simulink model "FBR25_model_4_rotating_tyres_with_ground_no_contact"  (R2026a)
settings: Solver=VariableStepAuto  StopTime=5
model workspace: external: MATLAB File /Users/janabauer/Desktop/LTS-test/models/FBR25forVD_DataFile1.m (data not in the file)
undefined symbols (not defined in the file or in its folder): smiData, X, Y, Z
libraries: sm_lib x832, nesl_utility x5, simulink x1
(part 13 of 13)

== system FBR25_model_4_rotating_tyres_with_ground_no_contact/FBR25_VD_1_RIGID/FBR25_VD_0300_STEERING_Computurtle_3_1_RIGID/FBR25_VD_33_00_1_RIGID/FBR25_VD_33_06_1_RIGID ==
  ReferenceFrame : sm_lib/Frames and Transforms/Reference Frame
  Solid : sm_lib/Body Elements/File Solid  ExtGeomFileName=FBR25-VD-33-06_Default_sldprt.STEP  UnitType=FromFile  ExtGeomFileUnits=m  StepReaderType=HEX  ExportConvexHullGeometry=off  InertiaType=Custom  BasedOnType=DensityFromFile  Density=1000  DensityUnits=kg/m^3  Mass=smiData.Solid(89).mass  MassUnits=kg  CenterOfMass=smiData.Solid(89).CoM  CenterOfMassUnits=mm  MomentsOfInertia=smiData.Solid(89).MoI  MomentsOfInertiaUnits=kg*mm^2  ProductsOfInertia=smiData.Solid(89).PoI  ProductsOfInertiaUnits=kg*mm^2  GraphicType=FromGeometry  MarkerShape=Sphere  MarkerSize=10  GraphicVisPropType=SimpleVisualProperties  GraphicDiffuseColor=smiData.Solid(89).color  GraphicOpacity=smiData.Solid(89).opacity  GraphicSpecularColor=[0.5 0.5 0.5 1.0]  GraphicAmbientColor=[0.15 0.15 0.15 1.0]  GraphicEmissiveColor=[0.0 0.0 0.0 1.0]  GraphicShininess=75  DoExposeReferenceFrame=on  SerializedFrames=<Frames/>
  F : PMIOPort  Side=Left
  connections:
  Solid/RConn1 -- ReferenceFrame/RConn1 -- F/RConn1

== system FBR25_model_4_rotating_tyres_with_ground_no_contact/FBR25_VD_1_RIGID/FBR25_VD_0300_STEERING_Computurtle_3_1_RIGID/FBR25_VD_33_00_1_RIGID/FBR25_VD_33_06_2_RIGID ==
  ReferenceFrame : sm_lib/Frames and Transforms/Reference Frame
  Solid : sm_lib/Body Elements/File Solid  ExtGeomFileName=FBR25-VD-33-06_Default_sldprt.STEP  UnitType=FromFile  ExtGeomFileUnits=m  StepReaderType=HEX  ExportConvexHullGeometry=off  InertiaType=Custom  BasedOnType=DensityFromFile  Density=1000  DensityUnits=kg/m^3  Mass=smiData.Solid(89).mass  MassUnits=kg  CenterOfMass=smiData.Solid(89).CoM  CenterOfMassUnits=mm  MomentsOfInertia=smiData.Solid(89).MoI  MomentsOfInertiaUnits=kg*mm^2  ProductsOfInertia=smiData.Solid(89).PoI  ProductsOfInertiaUnits=kg*mm^2  GraphicType=FromGeometry  MarkerShape=Sphere  MarkerSize=10  GraphicVisPropType=SimpleVisualProperties  GraphicDiffuseColor=smiData.Solid(89).color  GraphicOpacity=smiData.Solid(89).opacity  GraphicSpecularColor=[0.5 0.5 0.5 1.0]  GraphicAmbientColor=[0.15 0.15 0.15 1.0]  GraphicEmissiveColor=[0.0 0.0 0.0 1.0]  GraphicShininess=75  DoExposeReferenceFrame=on  SerializedFrames=<Frames/>
  F : PMIOPort  Side=Left
  connections:
  Solid/RConn1 -- ReferenceFrame/RConn1 -- F/RConn1

== system FBR25_model_4_rotating_tyres_with_ground_no_contact/FBR25_VD_1_RIGID/FBR25_VD_0300_STEERING_Computurtle_3_1_RIGID/FBR25_VD_33_00_1_RIGID/Part3_1_RIGID ==
  ReferenceFrame : sm_lib/Frames and Transforms/Reference Frame
  Solid : sm_lib/Body Elements/File Solid  ExtGeomFileName=Part3_Default_sldprt.STEP  UnitType=FromFile  ExtGeomFileUnits=m  StepReaderType=HEX  ExportConvexHullGeometry=off  InertiaType=Custom  BasedOnType=DensityFromFile  Density=1000  DensityUnits=kg/m^3  Mass=smiData.Solid(90).mass  MassUnits=kg  CenterOfMass=smiData.Solid(90).CoM  CenterOfMassUnits=mm  MomentsOfInertia=smiData.Solid(90).MoI  MomentsOfInertiaUnits=kg*mm^2  ProductsOfInertia=smiData.Solid(90).PoI  ProductsOfInertiaUnits=kg*mm^2  GraphicType=FromGeometry  MarkerShape=Sphere  MarkerSize=10  GraphicVisPropType=SimpleVisualProperties  GraphicDiffuseColor=smiData.Solid(90).color  GraphicOpacity=smiData.Solid(90).opacity  GraphicSpecularColor=[0.5 0.5 0.5 1.0]  GraphicAmbientColor=[0.15 0.15 0.15 1.0]  GraphicEmissiveColor=[0.0 0.0 0.0 1.0]  GraphicShininess=75  DoExposeReferenceFrame=on  SerializedFrames=<Frames/>
  F : PMIOPort  Side=Left
  connections:
  Solid/RConn1 -- ReferenceFrame/RConn1 -- F/RConn1

== system FBR25_model_4_rotating_tyres_with_ground_no_contact/FBR25_VD_1_RIGID/FBR25_VD_0300_STEERING_Computurtle_3_1_RIGID/FBR25_VD_33_00_1_RIGID/Part3_2_RIGID ==
  ReferenceFrame : sm_lib/Frames and Transforms/Reference Frame
  Solid : sm_lib/Body Elements/File Solid  ExtGeomFileName=Part3_Default_sldprt.STEP  UnitType=FromFile  ExtGeomFileUnits=m  StepReaderType=HEX  ExportConvexHullGeometry=off  InertiaType=Custom  BasedOnType=DensityFromFile  Density=1000  DensityUnits=kg/m^3  Mass=smiData.Solid(90).mass  MassUnits=kg  CenterOfMass=smiData.Solid(90).CoM  CenterOfMassUnits=mm  MomentsOfInertia=smiData.Solid(90).MoI  MomentsOfInertiaUnits=kg*mm^2  ProductsOfInertia=smiData.Solid(90).PoI  ProductsOfInertiaUnits=kg*mm^2  GraphicType=FromGeometry  MarkerShape=Sphere  MarkerSize=10  GraphicVisPropType=SimpleVisualProperties  GraphicDiffuseColor=smiData.Solid(90).color  GraphicOpacity=smiData.Solid(90).opacity  GraphicSpecularColor=[0.5 0.5 0.5 1.0]  GraphicAmbientColor=[0.15 0.15 0.15 1.0]  GraphicEmissiveColor=[0.0 0.0 0.0 1.0]  GraphicShininess=75  DoExposeReferenceFrame=on  SerializedFrames=<Frames/>
  F : PMIOPort  Side=Left
  connections:
  Solid/RConn1 -- ReferenceFrame/RConn1 -- F/RConn1

== system FBR25_model_4_rotating_tyres_with_ground_no_contact/FBR25_VD_1_RIGID/FBR25_VD_0300_STEERING_Computurtle_3_1_RIGID/FBR25_VD_33_00_1_RIGID/SPACER_M8_MISALIGNMENT_1_RIGID ==
  ReferenceFrame : sm_lib/Frames and Transforms/Reference Frame
  Solid : sm_lib/Body Elements/File Solid  ExtGeomFileName=SPACER - M8 MISALIGNMENT_Default_sldprt.STEP  UnitType=FromFile  ExtGeomFileUnits=m  StepReaderType=HEX  ExportConvexHullGeometry=off  InertiaType=Custom  BasedOnType=DensityFromFile  Density=1000  DensityUnits=kg/m^3  Mass=smiData.Solid(23).mass  MassUnits=kg  CenterOfMass=smiData.Solid(23).CoM  CenterOfMassUnits=mm  MomentsOfInertia=smiData.Solid(23).MoI  MomentsOfInertiaUnits=kg*mm^2  ProductsOfInertia=smiData.Solid(23).PoI  ProductsOfInertiaUnits=kg*mm^2  GraphicType=FromGeometry  MarkerShape=Sphere  MarkerSize=10  GraphicVisPropType=SimpleVisualProperties  GraphicDiffuseColor=smiData.Solid(23).color  GraphicOpacity=smiData.Solid(23).opacity  GraphicSpecularColor=[0.5 0.5 0.5 1.0]  GraphicAmbientColor=[0.15 0.15 0.15 1.0]  GraphicEmissiveColor=[0.0 0.0 0.0 1.0]  GraphicShininess=75  DoExposeReferenceFrame=on  SerializedFrames=<Frames/>
  F : PMIOPort  Side=Left
  connections:
  Solid/RConn1 -- ReferenceFrame/RConn1 -- F/RConn1

== system FBR25_model_4_rotating_tyres_with_ground_no_contact/FBR25_VD_1_RIGID/FBR25_VD_0300_STEERING_Computurtle_3_1_RIGID/FBR25_VD_33_00_1_RIGID/SPACER_M8_MISALIGNMENT_2_RIGID ==
  ReferenceFrame : sm_lib/Frames and Transforms/Reference Frame
  Solid : sm_lib/Body Elements/File Solid  ExtGeomFileName=SPACER - M8 MISALIGNMENT_Default_sldprt.STEP  UnitType=FromFile  ExtGeomFileUnits=m  StepReaderType=HEX  ExportConvexHullGeometry=off  InertiaType=Custom  BasedOnType=DensityFromFile  Density=1000  DensityUnits=kg/m^3  Mass=smiData.Solid(23).mass  MassUnits=kg  CenterOfMass=smiData.Solid(23).CoM  CenterOfMassUnits=mm  MomentsOfInertia=smiData.Solid(23).MoI  MomentsOfInertiaUnits=kg*mm^2  ProductsOfInertia=smiData.Solid(23).PoI  ProductsOfInertiaUnits=kg*mm^2  GraphicType=FromGeometry  MarkerShape=Sphere  MarkerSize=10  GraphicVisPropType=SimpleVisualProperties  GraphicDiffuseColor=smiData.Solid(23).color  GraphicOpacity=smiData.Solid(23).opacity  GraphicSpecularColor=[0.5 0.5 0.5 1.0]  GraphicAmbientColor=[0.15 0.15 0.15 1.0]  GraphicEmissiveColor=[0.0 0.0 0.0 1.0]  GraphicShininess=75  DoExposeReferenceFrame=on  SerializedFrames=<Frames/>
  F : PMIOPort  Side=Left
  connections:
  Solid/RConn1 -- ReferenceFrame/RConn1 -- F/RConn1

== system FBR25_model_4_rotating_tyres_with_ground_no_contact/FBR25_VD_1_RIGID/FBR25_VD_0300_STEERING_Computurtle_3_1_RIGID/FBR25_VD_33_00_1_RIGID/SPACER_M8_MISALIGNMENT_3_RIGID ==
  ReferenceFrame : sm_lib/Frames and Transforms/Reference Frame
  Solid : sm_lib/Body Elements/File Solid  ExtGeomFileName=SPACER - M8 MISALIGNMENT_Default_sldprt.STEP  UnitType=FromFile  ExtGeomFileUnits=m  StepReaderType=HEX  ExportConvexHullGeometry=off  InertiaType=Custom  BasedOnType=DensityFromFile  Density=1000  DensityUnits=kg/m^3  Mass=smiData.Solid(23).mass  MassUnits=kg  CenterOfMass=smiData.Solid(23).CoM  CenterOfMassUnits=mm  MomentsOfInertia=smiData.Solid(23).MoI  MomentsOfInertiaUnits=kg*mm^2  ProductsOfInertia=smiData.Solid(23).PoI  ProductsOfInertiaUnits=kg*mm^2  GraphicType=FromGeometry  MarkerShape=Sphere  MarkerSize=10  GraphicVisPropType=SimpleVisualProperties  GraphicDiffuseColor=smiData.Solid(23).color  GraphicOpacity=smiData.Solid(23).opacity  GraphicSpecularColor=[0.5 0.5 0.5 1.0]  GraphicAmbientColor=[0.15 0.15 0.15 1.0]  GraphicEmissiveColor=[0.0 0.0 0.0 1.0]  GraphicShininess=75  DoExposeReferenceFrame=on  SerializedFrames=<Frames/>
  F : PMIOPort  Side=Left
  connections:
  Solid/RConn1 -- ReferenceFrame/RConn1 -- F/RConn1

== system FBR25_model_4_rotating_tyres_with_ground_no_contact/FBR25_VD_1_RIGID/FBR25_VD_0300_STEERING_Computurtle_3_1_RIGID/FBR25_VD_33_00_1_RIGID/SPACER_M8_MISALIGNMENT_4_RIGID ==
  ReferenceFrame : sm_lib/Frames and Transforms/Reference Frame
  Solid : sm_lib/Body Elements/File Solid  ExtGeomFileName=SPACER - M8 MISALIGNMENT_Default_sldprt.STEP  UnitType=FromFile  ExtGeomFileUnits=m  StepReaderType=HEX  ExportConvexHullGeometry=off  InertiaType=Custom  BasedOnType=DensityFromFile  Density=1000  DensityUnits=kg/m^3  Mass=smiData.Solid(23).mass  MassUnits=kg  CenterOfMass=smiData.Solid(23).CoM  CenterOfMassUnits=mm  MomentsOfInertia=smiData.Solid(23).MoI  MomentsOfInertiaUnits=kg*mm^2  ProductsOfInertia=smiData.Solid(23).PoI  ProductsOfInertiaUnits=kg*mm^2  GraphicType=FromGeometry  MarkerShape=Sphere  MarkerSize=10  GraphicVisPropType=SimpleVisualProperties  GraphicDiffuseColor=smiData.Solid(23).color  GraphicOpacity=smiData.Solid(23).opacity  GraphicSpecularColor=[0.5 0.5 0.5 1.0]  GraphicAmbientColor=[0.15 0.15 0.15 1.0]  GraphicEmissiveColor=[0.0 0.0 0.0 1.0]  GraphicShininess=75  DoExposeReferenceFrame=on  SerializedFrames=<Frames/>
  F : PMIOPort  Side=Left
  connections:
  Solid/RConn1 -- ReferenceFrame/RConn1 -- F/RConn1

== system FBR25_model_4_rotating_tyres_with_ground_no_contact/FBR25_VD_1_RIGID/FBR25_VD_0000_WISHBONES_1_RIGID/FBR25_VD_0010_WB_F_U_1_RIGID/FBR25_VD_00_14_NH_01_1_RIGID/FBR25_VD_00_14_NH_01_ball_1_RIGID ==
  ReferenceFrame : sm_lib/Frames and Transforms/Reference Frame
  Solid : sm_lib/Body Elements/File Solid  ExtGeomFileName=FBR25-VD-00-14-NH-01 ball_Default_sldprt.STEP  UnitType=FromFile  ExtGeomFileUnits=m  StepReaderType=HEX  ExportConvexHullGeometry=off  InertiaType=Custom  BasedOnType=DensityFromFile  Density=1000  DensityUnits=kg/m^3  Mass=smiData.Solid(30).mass  MassUnits=kg  CenterOfMass=smiData.Solid(30).CoM  CenterOfMassUnits=mm  MomentsOfInertia=smiData.Solid(30).MoI  MomentsOfInertiaUnits=kg*mm^2  ProductsOfInertia=smiData.Solid(30).PoI  ProductsOfInertiaUnits=kg*mm^2  GraphicType=FromGeometry  MarkerShape=Sphere  MarkerSize=10  GraphicVisPropType=SimpleVisualProperties  GraphicDiffuseColor=smiData.Solid(30).color  GraphicOpacity=smiData.Solid(30).opacity  GraphicSpecularColor=[0.5 0.5 0.5 1.0]  GraphicAmbientColor=[0.15 0.15 0.15 1.0]  GraphicEmissiveColor=[0.0 0.0 0.0 1.0]  GraphicShininess=75  DoExposeReferenceFrame=on  SerializedFrames=<Frames/>
  F : PMIOPort  Side=Left
  connections:
  Solid/RConn1 -- ReferenceFrame/RConn1 -- F/RConn1

== system FBR25_model_4_rotating_tyres_with_ground_no_contact/FBR25_VD_1_RIGID/FBR25_VD_0000_WISHBONES_1_RIGID/FBR25_VD_0010_WB_F_U_1_RIGID/FBR25_VD_00_14_NH_01_1_RIGID/FBR25_VD_00_14_NH_01_casing_1_RIGID ==
  ReferenceFrame : sm_lib/Frames and Transforms/Reference Frame
  Solid : sm_lib/Body Elements/File Solid  ExtGeomFileName=FBR25-VD-00-14-NH-01 casing_Default_sldprt.STEP  UnitType=FromFile  ExtGeomFileUnits=m  StepReaderType=HEX  ExportConvexHullGeometry=off  InertiaType=Custom  BasedOnType=DensityFromFile  Density=1000  DensityUnits=kg/m^3  Mass=smiData.Solid(31).mass  MassUnits=kg  CenterOfMass=smiData.Solid(31).CoM  CenterOfMassUnits=mm  MomentsOfInertia=smiData.Solid(31).MoI  MomentsOfInertiaUnits=kg*mm^2  ProductsOfInertia=smiData.Solid(31).PoI  ProductsOfInertiaUnits=kg*mm^2  GraphicType=FromGeometry  MarkerShape=Sphere  MarkerSize=10  GraphicVisPropType=SimpleVisualProperties  GraphicDiffuseColor=smiData.Solid(31).color  GraphicOpacity=smiData.Solid(31).opacity  GraphicSpecularColor=[0.5 0.5 0.5 1.0]  GraphicAmbientColor=[0.15 0.15 0.15 1.0]  GraphicEmissiveColor=[0.0 0.0 0.0 1.0]  GraphicShininess=75  DoExposeReferenceFrame=on  SerializedFrames=<Frames/>
  F : PMIOPort  Side=Left
  connections:
  Solid/RConn1 -- ReferenceFrame/RConn1 -- F/RConn1

== system FBR25_model_4_rotating_tyres_with_ground_no_contact/FBR25_VD_1_RIGID/FBR25_VD_0000_WISHBONES_1_RIGID/FBR25_VD_0020_1_RIGID/FBR25_VD_00_24_NH_01_1_RIGID/FBR25_VD_00_24_NH_01_ball_1_RIGID ==
  ReferenceFrame : sm_lib/Frames and Transforms/Reference Frame
  Solid : sm_lib/Body Elements/File Solid  ExtGeomFileName=FBR25-VD-00-24-NH-01 - ball_Default_sldprt.STEP  UnitType=FromFile  ExtGeomFileUnits=m  StepReaderType=HEX  ExportConvexHullGeometry=off  InertiaType=Custom  BasedOnType=DensityFromFile  Density=1000  DensityUnits=kg/m^3  Mass=smiData.Solid(49).mass  MassUnits=kg  CenterOfMass=smiData.Solid(49).CoM  CenterOfMassUnits=mm  MomentsOfInertia=smiData.Solid(49).MoI  MomentsOfInertiaUnits=kg*mm^2  ProductsOfInertia=smiData.Solid(49).PoI  ProductsOfInertiaUnits=kg*mm^2  GraphicType=FromGeometry  MarkerShape=Sphere  MarkerSize=10  GraphicVisPropType=SimpleVisualProperties  GraphicDiffuseColor=smiData.Solid(49).color  GraphicOpacity=smiData.Solid(49).opacity  GraphicSpecularColor=[0.5 0.5 0.5 1.0]  GraphicAmbientColor=[0.15 0.15 0.15 1.0]  GraphicEmissiveColor=[0.0 0.0 0.0 1.0]  GraphicShininess=75  DoExposeReferenceFrame=on  SerializedFrames=<Frames/>
  F : PMIOPort  Side=Left
  connections:
  Solid/RConn1 -- ReferenceFrame/RConn1 -- F/RConn1

== system FBR25_model_4_rotating_tyres_with_ground_no_contact/FBR25_VD_1_RIGID/FBR25_VD_0000_WISHBONES_1_RIGID/FBR25_VD_0020_1_RIGID/FBR25_VD_00_24_NH_01_1_RIGID/FBR25_VD_00_24_NH_01_casing_1_RIGID ==
  ReferenceFrame : sm_lib/Frames and Transforms/Reference Frame
  Solid : sm_lib/Body Elements/File Solid  ExtGeomFileName=FBR25-VD-00-24-NH-01 - casing_Default_sldprt.STEP  UnitType=FromFile  ExtGeomFileUnits=m  StepReaderType=HEX  ExportConvexHullGeometry=off  InertiaType=Custom  BasedOnType=DensityFromFile  Density=1000  DensityUnits=kg/m^3  Mass=smiData.Solid(48).mass  MassUnits=kg  CenterOfMass=smiData.Solid(48).CoM  CenterOfMassUnits=mm  MomentsOfInertia=smiData.Solid(48).MoI  MomentsOfInertiaUnits=kg*mm^2  ProductsOfInertia=smiData.Solid(48).PoI  ProductsOfInertiaUnits=kg*mm^2  GraphicType=FromGeometry  MarkerShape=Sphere  MarkerSize=10  GraphicVisPropType=SimpleVisualProperties  GraphicDiffuseColor=smiData.Solid(48).color  GraphicOpacity=smiData.Solid(48).opacity  GraphicSpecularColor=[0.5 0.5 0.5 1.0]  GraphicAmbientColor=[0.15 0.15 0.15 1.0]  GraphicEmissiveColor=[0.0 0.0 0.0 1.0]  GraphicShininess=75  DoExposeReferenceFrame=on  SerializedFrames=<Frames/>
  F : PMIOPort  Side=Left
  connections:
  Solid/RConn1 -- ReferenceFrame/RConn1 -- F/RConn1

== system FBR25_model_4_rotating_tyres_with_ground_no_contact/FBR25_VD_1_RIGID/FBR25_VD_0000_WISHBONES_1_RIGID/FBR25_VD_0020_1_RIGID/MirrorFBR25_VD_00_24_NH_01_2_RIGID/MirrorFBR25_VD_00_24_NH_01_ball_1_RIGID ==
  ReferenceFrame : sm_lib/Frames and Transforms/Reference Frame
  Solid : sm_lib/Body Elements/File Solid  ExtGeomFileName=MirrorFBR25-VD-00-24-NH-01 - ball_Default_sldprt.STEP  UnitType=FromFile  ExtGeomFileUnits=m  StepReaderType=HEX  ExportConvexHullGeometry=off  InertiaType=Custom  BasedOnType=DensityFromFile  Density=1000  DensityUnits=kg/m^3  Mass=smiData.Solid(54).mass  MassUnits=kg  CenterOfMass=smiData.Solid(54).CoM  CenterOfMassUnits=mm  MomentsOfInertia=smiData.Solid(54).MoI  MomentsOfInertiaUnits=kg*mm^2  ProductsOfInertia=smiData.Solid(54).PoI  ProductsOfInertiaUnits=kg*mm^2  GraphicType=FromGeometry  MarkerShape=Sphere  MarkerSize=10  GraphicVisPropType=SimpleVisualProperties  GraphicDiffuseColor=smiData.Solid(54).color  GraphicOpacity=smiData.Solid(54).opacity  GraphicSpecularColor=[0.5 0.5 0.5 1.0]  GraphicAmbientColor=[0.15 0.15 0.15 1.0]  GraphicEmissiveColor=[0.0 0.0 0.0 1.0]  GraphicShininess=75  DoExposeReferenceFrame=on  SerializedFrames=<Frames/>
  F : PMIOPort  Side=Left
  connections:
  Solid/RConn1 -- ReferenceFrame/RConn1 -- F/RConn1

== system FBR25_model_4_rotating_tyres_with_ground_no_contact/FBR25_VD_1_RIGID/FBR25_VD_0000_WISHBONES_1_RIGID/FBR25_VD_0020_1_RIGID/MirrorFBR25_VD_00_24_NH_01_2_RIGID/MirrorFBR25_VD_00_24_NH_01_casing_1_RIGID ==
  ReferenceFrame : sm_lib/Frames and Transforms/Reference Frame
  Solid : sm_lib/Body Elements/File Solid  ExtGeomFileName=MirrorFBR25-VD-00-24-NH-01 - casing_Default_sldprt.STEP  UnitType=FromFile  ExtGeomFileUnits=m  StepReaderType=HEX  ExportConvexHullGeometry=off  InertiaType=Custom  BasedOnType=DensityFromFile  Density=1000  DensityUnits=kg/m^3  Mass=smiData.Solid(53).mass  MassUnits=kg  CenterOfMass=smiData.Solid(53).CoM  CenterOfMassUnits=mm  MomentsOfInertia=smiData.Solid(53).MoI  MomentsOfInertiaUnits=kg*mm^2  ProductsOfInertia=smiData.Solid(53).PoI  ProductsOfInertiaUnits=kg*mm^2  GraphicType=FromGeometry  MarkerShape=Sphere  MarkerSize=10  GraphicVisPropType=SimpleVisualProperties  GraphicDiffuseColor=smiData.Solid(53).color  GraphicOpacity=smiData.Solid(53).opacity  GraphicSpecularColor=[0.5 0.5 0.5 1.0]  GraphicAmbientColor=[0.15 0.15 0.15 1.0]  GraphicEmissiveColor=[0.0 0.0 0.0 1.0]  GraphicShininess=75  DoExposeReferenceFrame=on  SerializedFrames=<Frames/>
  F : PMIOPort  Side=Left
  connections:
  Solid/RConn1 -- ReferenceFrame/RConn1 -- F/RConn1

== system FBR25_model_4_rotating_tyres_with_ground_no_contact/FBR25_VD_1_RIGID/FBR25_VD_0000_WISHBONES_1_RIGID/FBR25_VD_0060_2_RIGID/FBR25_VD_00_64_NH_01_1_RIGID/FBR25_VD_00_64_NH_01_ball_1_RIGID ==
  ReferenceFrame : sm_lib/Frames and Transforms/Reference Frame
  Solid : sm_lib/Body Elements/File Solid  ExtGeomFileName=FBR25-VD-00-64-NH-01 ball_Default_sldprt.STEP  UnitType=FromFile  ExtGeomFileUnits=m  StepReaderType=HEX  ExportConvexHullGeometry=off  InertiaType=Custom  BasedOnType=DensityFromFile  Density=1000  DensityUnits=kg/m^3  Mass=smiData.Solid(41).mass  MassUnits=kg  CenterOfMass=smiData.Solid(41).CoM  CenterOfMassUnits=mm  MomentsOfInertia=smiData.Solid(41).MoI  MomentsOfInertiaUnits=kg*mm^2  ProductsOfInertia=smiData.Solid(41).PoI  ProductsOfInertiaUnits=kg*mm^2  GraphicType=FromGeometry  MarkerShape=Sphere  MarkerSize=10  GraphicVisPropType=SimpleVisualProperties  GraphicDiffuseColor=smiData.Solid(41).color  GraphicOpacity=smiData.Solid(41).opacity  GraphicSpecularColor=[0.5 0.5 0.5 1.0]  GraphicAmbientColor=[0.15 0.15 0.15 1.0]  GraphicEmissiveColor=[0.0 0.0 0.0 1.0]  GraphicShininess=75  DoExposeReferenceFrame=on  SerializedFrames=<Frames/>
  F : PMIOPort  Side=Left
  connections:
  Solid/RConn1 -- ReferenceFrame/RConn1 -- F/RConn1

== system FBR25_model_4_rotating_tyres_with_ground_no_contact/FBR25_VD_1_RIGID/FBR25_VD_0000_WISHBONES_1_RIGID/FBR25_VD_0060_2_RIGID/FBR25_VD_00_64_NH_01_1_RIGID/FBR25_VD_00_64_NH_01_casing_1_RIGID ==
  ReferenceFrame : sm_lib/Frames and Transforms/Reference Frame
  Solid : sm_lib/Body Elements/File Solid  ExtGeomFileName=FBR25-VD-00-64-NH-01 casing_Default_sldprt.STEP  UnitType=FromFile  ExtGeomFileUnits=m  StepReaderType=HEX  ExportConvexHullGeometry=off  InertiaType=Custom  BasedOnType=DensityFromFile  Density=1000  DensityUnits=kg/m^3  Mass=smiData.Solid(42).mass  MassUnits=kg  CenterOfMass=smiData.Solid(42).CoM  CenterOfMassUnits=mm  MomentsOfInertia=smiData.Solid(42).MoI  MomentsOfInertiaUnits=kg*mm^2  ProductsOfInertia=smiData.Solid(42).PoI  ProductsOfInertiaUnits=kg*mm^2  GraphicType=FromGeometry  MarkerShape=Sphere  MarkerSize=10  GraphicVisPropType=SimpleVisualProperties  GraphicDiffuseColor=smiData.Solid(42).color  GraphicOpacity=smiData.Solid(42).opacity  GraphicSpecularColor=[0.5 0.5 0.5 1.0]  GraphicAmbientColor=[0.15 0.15 0.15 1.0]  GraphicEmissiveColor=[0.0 0.0 0.0 1.0]  GraphicShininess=75  DoExposeReferenceFrame=on  SerializedFrames=<Frames/>
  F : PMIOPort  Side=Left
  connections:
  Solid/RConn1 -- ReferenceFrame/RConn1 -- F/RConn1

== system FBR25_model_4_rotating_tyres_with_ground_no_contact/FBR25_VD_1_RIGID/FBR25_VD_0000_WISHBONES_1_RIGID/FBR25_VD_0060_2_RIGID/FBR25_VD_00_64_NH_01_2_RIGID/FBR25_VD_00_64_NH_01_ball_1_RIGID ==
  ReferenceFrame : sm_lib/Frames and Transforms/Reference Frame
  Solid : sm_lib/Body Elements/File Solid  ExtGeomFileName=FBR25-VD-00-64-NH-01 ball_Default_sldprt.STEP  UnitType=FromFile  ExtGeomFileUnits=m  StepReaderType=HEX  ExportConvexHullGeometry=off  InertiaType=Custom  BasedOnType=DensityFromFile  Density=1000  DensityUnits=kg/m^3  Mass=smiData.Solid(41).mass  MassUnits=kg  CenterOfMass=smiData.Solid(41).CoM  CenterOfMassUnits=mm  MomentsOfInertia=smiData.Solid(41).MoI  MomentsOfInertiaUnits=kg*mm^2  ProductsOfInertia=smiData.Solid(41).PoI  ProductsOfInertiaUnits=kg*mm^2  GraphicType=FromGeometry  MarkerShape=Sphere  MarkerSize=10  GraphicVisPropType=SimpleVisualProperties  GraphicDiffuseColor=smiData.Solid(41).color  GraphicOpacity=smiData.Solid(41).opacity  GraphicSpecularColor=[0.5 0.5 0.5 1.0]  GraphicAmbientColor=[0.15 0.15 0.15 1.0]  GraphicEmissiveColor=[0.0 0.0 0.0 1.0]  GraphicShininess=75  DoExposeReferenceFrame=on  SerializedFrames=<Frames/>
  F : PMIOPort  Side=Left
  connections:
  Solid/RConn1 -- ReferenceFrame/RConn1 -- F/RConn1

== system FBR25_model_4_rotating_tyres_with_ground_no_contact/FBR25_VD_1_RIGID/FBR25_VD_0000_WISHBONES_1_RIGID/FBR25_VD_0060_2_RIGID/FBR25_VD_00_64_NH_01_2_RIGID/FBR25_VD_00_64_NH_01_casing_1_RIGID ==
  ReferenceFrame : sm_lib/Frames and Transforms/Reference Frame
  Solid : sm_lib/Body Elements/File Solid  ExtGeomFileName=FBR25-VD-00-64-NH-01 casing_Default_sldprt.STEP  UnitType=FromFile  ExtGeomFileUnits=m  StepReaderType=HEX  ExportConvexHullGeometry=off  InertiaType=Custom  BasedOnType=DensityFromFile  Density=1000  DensityUnits=kg/m^3  Mass=smiData.Solid(42).mass  MassUnits=kg  CenterOfMass=smiData.Solid(42).CoM  CenterOfMassUnits=mm  MomentsOfInertia=smiData.Solid(42).MoI  MomentsOfInertiaUnits=kg*mm^2  ProductsOfInertia=smiData.Solid(42).PoI  ProductsOfInertiaUnits=kg*mm^2  GraphicType=FromGeometry  MarkerShape=Sphere  MarkerSize=10  GraphicVisPropType=SimpleVisualProperties  GraphicDiffuseColor=smiData.Solid(42).color  GraphicOpacity=smiData.Solid(42).opacity  GraphicSpecularColor=[0.5 0.5 0.5 1.0]  GraphicAmbientColor=[0.15 0.15 0.15 1.0]  GraphicEmissiveColor=[0.0 0.0 0.0 1.0]  GraphicShininess=75  DoExposeReferenceFrame=on  SerializedFrames=<Frames/>
  F : PMIOPort  Side=Left
  connections:
  Solid/RConn1 -- ReferenceFrame/RConn1 -- F/RConn1

== system FBR25_model_4_rotating_tyres_with_ground_no_contact/FBR25_VD_1_RIGID/FBR25_VD_0000_WISHBONES_1_RIGID/FBR25_VD_0070_1_RIGID/FBR25_VD_00_24_NH_01_1_RIGID/FBR25_VD_00_24_NH_01_ball_1_RIGID ==
  ReferenceFrame : sm_lib/Frames and Transforms/Reference Frame
  Solid : sm_lib/Body Elements/File Solid  ExtGeomFileName=FBR25-VD-00-24-NH-01 - ball_Default_sldprt.STEP  UnitType=FromFile  ExtGeomFileUnits=m  StepReaderType=HEX  ExportConvexHullGeometry=off  InertiaType=Custom  BasedOnType=DensityFromFile  Density=1000  DensityUnits=kg/m^3  Mass=smiData.Solid(49).mass  MassUnits=kg  CenterOfMass=smiData.Solid(49).CoM  CenterOfMassUnits=mm  MomentsOfInertia=smiData.Solid(49).MoI  MomentsOfInertiaUnits=kg*mm^2  ProductsOfInertia=smiData.Solid(49).PoI  ProductsOfInertiaUnits=kg*mm^2  GraphicType=FromGeometry  MarkerShape=Sphere  MarkerSize=10  GraphicVisPropType=SimpleVisualProperties  GraphicDiffuseColor=smiData.Solid(49).color  GraphicOpacity=smiData.Solid(49).opacity  GraphicSpecularColor=[0.5 0.5 0.5 1.0]  GraphicAmbientColor=[0.15 0.15 0.15 1.0]  GraphicEmissiveColor=[0.0 0.0 0.0 1.0]  GraphicShininess=75  DoExposeReferenceFrame=on  SerializedFrames=<Frames/>
  F : PMIOPort  Side=Left
  connections:
  Solid/RConn1 -- ReferenceFrame/RConn1 -- F/RConn1

== system FBR25_model_4_rotating_tyres_with_ground_no_contact/FBR25_VD_1_RIGID/FBR25_VD_0000_WISHBONES_1_RIGID/FBR25_VD_0070_1_RIGID/FBR25_VD_00_24_NH_01_1_RIGID/FBR25_VD_00_24_NH_01_casing_1_RIGID ==
  ReferenceFrame : sm_lib/Frames and Transforms/Reference Frame
  Solid : sm_lib/Body Elements/File Solid  ExtGeomFileName=FBR25-VD-00-24-NH-01 - casing_Default_sldprt.STEP  UnitType=FromFile  ExtGeomFileUnits=m  StepReaderType=HEX  ExportConvexHullGeometry=off  InertiaType=Custom  BasedOnType=DensityFromFile  Density=1000  DensityUnits=kg/m^3  Mass=smiData.Solid(48).mass  MassUnits=kg  CenterOfMass=smiData.Solid(48).CoM  CenterOfMassUnits=mm  MomentsOfInertia=smiData.Solid(48).MoI  MomentsOfInertiaUnits=kg*mm^2  ProductsOfInertia=smiData.Solid(48).PoI  ProductsOfInertiaUnits=kg*mm^2  GraphicType=FromGeometry  MarkerShape=Sphere  MarkerSize=10  GraphicVisPropType=SimpleVisualProperties  GraphicDiffuseColor=smiData.Solid(48).color  GraphicOpacity=smiData.Solid(48).opacity  GraphicSpecularColor=[0.5 0.5 0.5 1.0]  GraphicAmbientColor=[0.15 0.15 0.15 1.0]  GraphicEmissiveColor=[0.0 0.0 0.0 1.0]  GraphicShininess=75  DoExposeReferenceFrame=on  SerializedFrames=<Frames/>
  F : PMIOPort  Side=Left
  connections:
  Solid/RConn1 -- ReferenceFrame/RConn1 -- F/RConn1

== system FBR25_model_4_rotating_tyres_with_ground_no_contact/FBR25_VD_1_RIGID/FBR25_VD_0000_WISHBONES_1_RIGID/FBR25_VD_0070_1_RIGID/MirrorFBR25_VD_00_24_NH_01_2_RIGID/MirrorFBR25_VD_00_24_NH_01_ball_1_RIGID ==
  ReferenceFrame : sm_lib/Frames and Transforms/Reference Frame
  Solid : sm_lib/Body Elements/File Solid  ExtGeomFileName=MirrorFBR25-VD-00-24-NH-01 - ball_Default_sldprt.STEP  UnitType=FromFile  ExtGeomFileUnits=m  StepReaderType=HEX  ExportConvexHullGeometry=off  InertiaType=Custom  BasedOnType=DensityFromFile  Density=1000  DensityUnits=kg/m^3  Mass=smiData.Solid(54).mass  MassUnits=kg  CenterOfMass=smiData.Solid(54).CoM  CenterOfMassUnits=mm  MomentsOfInertia=smiData.Solid(54).MoI  MomentsOfInertiaUnits=kg*mm^2  ProductsOfInertia=smiData.Solid(54).PoI  ProductsOfInertiaUnits=kg*mm^2  GraphicType=FromGeometry  MarkerShape=Sphere  MarkerSize=10  GraphicVisPropType=SimpleVisualProperties  GraphicDiffuseColor=smiData.Solid(54).color  GraphicOpacity=smiData.Solid(54).opacity  GraphicSpecularColor=[0.5 0.5 0.5 1.0]  GraphicAmbientColor=[0.15 0.15 0.15 1.0]  GraphicEmissiveColor=[0.0 0.0 0.0 1.0]  GraphicShininess=75  DoExposeReferenceFrame=on  SerializedFrames=<Frames/>
  F : PMIOPort  Side=Left
  connections:
  Solid/RConn1 -- ReferenceFrame/RConn1 -- F/RConn1

== system FBR25_model_4_rotating_tyres_with_ground_no_contact/FBR25_VD_1_RIGID/FBR25_VD_0000_WISHBONES_1_RIGID/FBR25_VD_0070_1_RIGID/MirrorFBR25_VD_00_24_NH_01_2_RIGID/MirrorFBR25_VD_00_24_NH_01_casing_1_RIGID ==
  ReferenceFrame : sm_lib/Frames and Transforms/Reference Frame
  Solid : sm_lib/Body Elements/File Solid  ExtGeomFileName=MirrorFBR25-VD-00-24-NH-01 - casing_Default_sldprt.STEP  UnitType=FromFile  ExtGeomFileUnits=m  StepReaderType=HEX  ExportConvexHullGeometry=off  InertiaType=Custom  BasedOnType=DensityFromFile  Density=1000  DensityUnits=kg/m^3  Mass=smiData.Solid(53).mass  MassUnits=kg  CenterOfMass=smiData.Solid(53).CoM  CenterOfMassUnits=mm  MomentsOfInertia=smiData.Solid(53).MoI  MomentsOfInertiaUnits=kg*mm^2  ProductsOfInertia=smiData.Solid(53).PoI  ProductsOfInertiaUnits=kg*mm^2  GraphicType=FromGeometry  MarkerShape=Sphere  MarkerSize=10  GraphicVisPropType=SimpleVisualProperties  GraphicDiffuseColor=smiData.Solid(53).color  GraphicOpacity=smiData.Solid(53).opacity  GraphicSpecularColor=[0.5 0.5 0.5 1.0]  GraphicAmbientColor=[0.15 0.15 0.15 1.0]  GraphicEmissiveColor=[0.0 0.0 0.0 1.0]  GraphicShininess=75  DoExposeReferenceFrame=on  SerializedFrames=<Frames/>
  F : PMIOPort  Side=Left
  connections:
  Solid/RConn1 -- ReferenceFrame/RConn1 -- F/RConn1

== system FBR25_model_4_rotating_tyres_with_ground_no_contact/FBR25_VD_1_RIGID/FBR25_VD_0300_STEERING_Computurtle_3_1_RIGID/FBR25_VD_32_00_1_RIGID/FBR25_VD_32_02_3_RIGID/UJ_BALL_1_RIGID ==
  ReferenceFrame : sm_lib/Frames and Transforms/Reference Frame
  Solid : sm_lib/Body Elements/File Solid  ExtGeomFileName=UJ - BALL_Default_sldprt.STEP  UnitType=FromFile  ExtGeomFileUnits=m  StepReaderType=HEX  ExportConvexHullGeometry=off  InertiaType=Custom  BasedOnType=DensityFromFile  Density=1000  DensityUnits=kg/m^3  Mass=smiData.Solid(83).mass  MassUnits=kg  CenterOfMass=smiData.Solid(83).CoM  CenterOfMassUnits=in  MomentsOfInertia=smiData.Solid(83).MoI  MomentsOfInertiaUnits=kg*in^2  ProductsOfInertia=smiData.Solid(83).PoI  ProductsOfInertiaUnits=kg*in^2  GraphicType=FromGeometry  MarkerShape=Sphere  MarkerSize=10  GraphicVisPropType=SimpleVisualProperties  GraphicDiffuseColor=smiData.Solid(83).color  GraphicOpacity=smiData.Solid(83).opacity  GraphicSpecularColor=[0.5 0.5 0.5 1.0]  GraphicAmbientColor=[0.15 0.15 0.15 1.0]  GraphicEmissiveColor=[0.0 0.0 0.0 1.0]  GraphicShininess=75  DoExposeReferenceFrame=on  SerializedFrames=<Frames/>
  F : PMIOPort  Side=Left
  connections:
  Solid/RConn1 -- ReferenceFrame/RConn1 -- F/RConn1

== system FBR25_model_4_rotating_tyres_with_ground_no_contact/FBR25_VD_1_RIGID/FBR25_VD_0300_STEERING_Computurtle_3_1_RIGID/FBR25_VD_32_00_1_RIGID/FBR25_VD_32_02_3_RIGID/UJ_HALF_INCH_LOWER_1_RIGID ==
  ReferenceFrame : sm_lib/Frames and Transforms/Reference Frame
  Solid : sm_lib/Body Elements/File Solid  ExtGeomFileName=UJ - HALF INCH LOWER_Default_sldprt.STEP  UnitType=FromFile  ExtGeomFileUnits=m  StepReaderType=HEX  ExportConvexHullGeometry=off  InertiaType=Custom  BasedOnType=DensityFromFile  Density=1000  DensityUnits=kg/m^3  Mass=smiData.Solid(82).mass  MassUnits=kg  CenterOfMass=smiData.Solid(82).CoM  CenterOfMassUnits=in  MomentsOfInertia=smiData.Solid(82).MoI  MomentsOfInertiaUnits=kg*in^2  ProductsOfInertia=smiData.Solid(82).PoI  ProductsOfInertiaUnits=kg*in^2  GraphicType=FromGeometry  MarkerShape=Sphere  MarkerSize=10  GraphicVisPropType=SimpleVisualProperties  GraphicDiffuseColor=smiData.Solid(82).color  GraphicOpacity=smiData.Solid(82).opacity  GraphicSpecularColor=[0.5 0.5 0.5 1.0]  GraphicAmbientColor=[0.15 0.15 0.15 1.0]  GraphicEmissiveColor=[0.0 0.0 0.0 1.0]  GraphicShininess=75  DoExposeReferenceFrame=on  SerializedFrames=<Frames/>
  F : PMIOPort  Side=Left
  connections:
  Solid/RConn1 -- ReferenceFrame/RConn1 -- F/RConn1

== system FBR25_model_4_rotating_tyres_with_ground_no_contact/FBR25_VD_1_RIGID/FBR25_VD_0300_STEERING_Computurtle_3_1_RIGID/FBR25_VD_32_00_1_RIGID/FBR25_VD_32_02_3_RIGID/UJ_HALF_INCH_UPPER_1_RIGID ==
  ReferenceFrame : sm_lib/Frames and Transforms/Reference Frame
  Solid : sm_lib/Body Elements/File Solid  ExtGeomFileName="UJ  - HALF INCH UPPER_Default_sldprt.STEP"  UnitType=FromFile  ExtGeomFileUnits=m  StepReaderType=HEX  ExportConvexHullGeometry=off  InertiaType=Custom  BasedOnType=DensityFromFile  Density=1000  DensityUnits=kg/m^3  Mass=smiData.Solid(81).mass  MassUnits=kg  CenterOfMass=smiData.Solid(81).CoM  CenterOfMassUnits=in  MomentsOfInertia=smiData.Solid(81).MoI  MomentsOfInertiaUnits=kg*in^2  ProductsOfInertia=smiData.Solid(81).PoI  ProductsOfInertiaUnits=kg*in^2  GraphicType=FromGeometry  MarkerShape=Sphere  MarkerSize=10  GraphicVisPropType=SimpleVisualProperties  GraphicDiffuseColor=smiData.Solid(81).color  GraphicOpacity=smiData.Solid(81).opacity  GraphicSpecularColor=[0.5 0.5 0.5 1.0]  GraphicAmbientColor=[0.15 0.15 0.15 1.0]  GraphicEmissiveColor=[0.0 0.0 0.0 1.0]  GraphicShininess=75  DoExposeReferenceFrame=on  SerializedFrames=<Frames/>
  F : PMIOPort  Side=Left
  connections:
  Solid/RConn1 -- ReferenceFrame/RConn1 -- F/RConn1

== system FBR25_model_4_rotating_tyres_with_ground_no_contact/FBR25_VD_1_RIGID/FBR25_VD_0300_STEERING_Computurtle_3_1_RIGID/FBR25_VD_32_00_1_RIGID/FBR25_VD_32_02_4_RIGID/UJ_BALL_1_RIGID ==
  ReferenceFrame : sm_lib/Frames and Transforms/Reference Frame
  Solid : sm_lib/Body Elements/File Solid  ExtGeomFileName=UJ - BALL_Default_sldprt.STEP  UnitType=FromFile  ExtGeomFileUnits=m  StepReaderType=HEX  ExportConvexHullGeometry=off  InertiaType=Custom  BasedOnType=DensityFromFile  Density=1000  DensityUnits=kg/m^3  Mass=smiData.Solid(83).mass  MassUnits=kg  CenterOfMass=smiData.Solid(83).CoM  CenterOfMassUnits=in  MomentsOfInertia=smiData.Solid(83).MoI  MomentsOfInertiaUnits=kg*in^2  ProductsOfInertia=smiData.Solid(83).PoI  ProductsOfInertiaUnits=kg*in^2  GraphicType=FromGeometry  MarkerShape=Sphere  MarkerSize=10  GraphicVisPropType=SimpleVisualProperties  GraphicDiffuseColor=smiData.Solid(83).color  GraphicOpacity=smiData.Solid(83).opacity  GraphicSpecularColor=[0.5 0.5 0.5 1.0]  GraphicAmbientColor=[0.15 0.15 0.15 1.0]  GraphicEmissiveColor=[0.0 0.0 0.0 1.0]  GraphicShininess=75  DoExposeReferenceFrame=on  SerializedFrames=<Frames/>
  F : PMIOPort  Side=Left
  connections:
  Solid/RConn1 -- ReferenceFrame/RConn1 -- F/RConn1

== system FBR25_model_4_rotating_tyres_with_ground_no_contact/FBR25_VD_1_RIGID/FBR25_VD_0300_STEERING_Computurtle_3_1_RIGID/FBR25_VD_32_00_1_RIGID/FBR25_VD_32_02_4_RIGID/UJ_HALF_INCH_LOWER_1_RIGID ==
  ReferenceFrame : sm_lib/Frames and Transforms/Reference Frame
  Solid : sm_lib/Body Elements/File Solid  ExtGeomFileName=UJ - HALF INCH LOWER_Default_sldprt.STEP  UnitType=FromFile  ExtGeomFileUnits=m  StepReaderType=HEX  ExportConvexHullGeometry=off  InertiaType=Custom  BasedOnType=DensityFromFile  Density=1000  DensityUnits=kg/m^3  Mass=smiData.Solid(82).mass  MassUnits=kg  CenterOfMass=smiData.Solid(82).CoM  CenterOfMassUnits=in  MomentsOfInertia=smiData.Solid(82).MoI  MomentsOfInertiaUnits=kg*in^2  ProductsOfInertia=smiData.Solid(82).PoI  ProductsOfInertiaUnits=kg*in^2  GraphicType=FromGeometry  MarkerShape=Sphere  MarkerSize=10  GraphicVisPropType=SimpleVisualProperties  GraphicDiffuseColor=smiData.Solid(82).color  GraphicOpacity=smiData.Solid(82).opacity  GraphicSpecularColor=[0.5 0.5 0.5 1.0]  GraphicAmbientColor=[0.15 0.15 0.15 1.0]  GraphicEmissiveColor=[0.0 0.0 0.0 1.0]  GraphicShininess=75  DoExposeReferenceFrame=on  SerializedFrames=<Frames/>
  F : PMIOPort  Side=Left
  connections:
  Solid/RConn1 -- ReferenceFrame/RConn1 -- F/RConn1

== system FBR25_model_4_rotating_tyres_with_ground_no_contact/FBR25_VD_1_RIGID/FBR25_VD_0300_STEERING_Computurtle_3_1_RIGID/FBR25_VD_32_00_1_RIGID/FBR25_VD_32_02_4_RIGID/UJ_HALF_INCH_UPPER_1_RIGID ==
  ReferenceFrame : sm_lib/Frames and Transforms/Reference Frame
  Solid : sm_lib/Body Elements/File Solid  ExtGeomFileName="UJ  - HALF INCH UPPER_Default_sldprt.STEP"  UnitType=FromFile  ExtGeomFileUnits=m  StepReaderType=HEX  ExportConvexHullGeometry=off  InertiaType=Custom  BasedOnType=DensityFromFile  Density=1000  DensityUnits=kg/m^3  Mass=smiData.Solid(81).mass  MassUnits=kg  CenterOfMass=smiData.Solid(81).CoM  CenterOfMassUnits=in  MomentsOfInertia=smiData.Solid(81).MoI  MomentsOfInertiaUnits=kg*in^2  ProductsOfInertia=smiData.Solid(81).PoI  ProductsOfInertiaUnits=kg*in^2  GraphicType=FromGeometry  MarkerShape=Sphere  MarkerSize=10  GraphicVisPropType=SimpleVisualProperties  GraphicDiffuseColor=smiData.Solid(81).color  GraphicOpacity=smiData.Solid(81).opacity  GraphicSpecularColor=[0.5 0.5 0.5 1.0]  GraphicAmbientColor=[0.15 0.15 0.15 1.0]  GraphicEmissiveColor=[0.0 0.0 0.0 1.0]  GraphicShininess=75  DoExposeReferenceFrame=on  SerializedFrames=<Frames/>
  F : PMIOPort  Side=Left
  connections:
  Solid/RConn1 -- ReferenceFrame/RConn1 -- F/RConn1

== system FBR25_model_4_rotating_tyres_with_ground_no_contact/FBR25_VD_1_RIGID/FBR25_VD_0300_STEERING_Computurtle_3_1_RIGID/FBR25_VD_33_00_1_RIGID/FBR25_VD_33_01_1_RIGID/PART_STEERING_RACK_BODY_with_added_points_1_RIGID ==
  ReferenceFrame : sm_lib/Frames and Transforms/Reference Frame
  Solid : sm_lib/Body Elements/File Solid  ExtGeomFileName=PART - STEERING RACK BODY with added points_Default_sldprt.STEP  UnitType=FromFile  ExtGeomFileUnits=m  StepReaderType=HEX  ExportConvexHullGeometry=off  InertiaType=Custom  BasedOnType=DensityFromFile  Density=1000  DensityUnits=kg/m^3  Mass=smiData.Solid(91).mass  MassUnits=kg  CenterOfMass=smiData.Solid(91).CoM  CenterOfMassUnits=mm  MomentsOfInertia=smiData.Solid(91).MoI  MomentsOfInertiaUnits=kg*mm^2  ProductsOfInertia=smiData.Solid(91).PoI  ProductsOfInertiaUnits=kg*mm^2  GraphicType=FromGeometry  MarkerShape=Sphere  MarkerSize=10  GraphicVisPropType=SimpleVisualProperties  GraphicDiffuseColor=smiData.Solid(91).color  GraphicOpacity=smiData.Solid(91).opacity  GraphicSpecularColor=[0.5 0.5 0.5 1.0]  GraphicAmbientColor=[0.15 0.15 0.15 1.0]  GraphicEmissiveColor=[0.0 0.0 0.0 1.0]  GraphicShininess=75  DoExposeReferenceFrame=on  SerializedFrames=<Frames/>
  F : PMIOPort  Side=Left
  connections:
  Solid/RConn1 -- ReferenceFrame/RConn1 -- F/RConn1

== system FBR25_model_4_rotating_tyres_with_ground_no_contact/FBR25_VD_1_RIGID/FBR25_VD_0300_STEERING_Computurtle_3_1_RIGID/FBR25_VD_33_00_1_RIGID/FBR25_VD_33_01_1_RIGID/PART_STEERING_RACK_MOUNT_with_added_points_1_RIGID ==
  ReferenceFrame : sm_lib/Frames and Transforms/Reference Frame
  Solid : sm_lib/Body Elements/File Solid  ExtGeomFileName=PART - STEERING RACK MOUNT with added points_Default_sldprt.STEP  UnitType=FromFile  ExtGeomFileUnits=m  StepReaderType=HEX  ExportConvexHullGeometry=off  InertiaType=Custom  BasedOnType=DensityFromFile  Density=1000  DensityUnits=kg/m^3  Mass=smiData.Solid(92).mass  MassUnits=kg  CenterOfMass=smiData.Solid(92).CoM  CenterOfMassUnits=mm  MomentsOfInertia=smiData.Solid(92).MoI  MomentsOfInertiaUnits=kg*mm^2  ProductsOfInertia=smiData.Solid(92).PoI  ProductsOfInertiaUnits=kg*mm^2  GraphicType=FromGeometry  MarkerShape=Sphere  MarkerSize=10  GraphicVisPropType=SimpleVisualProperties  GraphicDiffuseColor=smiData.Solid(92).color  GraphicOpacity=smiData.Solid(92).opacity  GraphicSpecularColor=[0.5 0.5 0.5 1.0]  GraphicAmbientColor=[0.15 0.15 0.15 1.0]  GraphicEmissiveColor=[0.0 0.0 0.0 1.0]  GraphicShininess=75  DoExposeReferenceFrame=on  SerializedFrames=<Frames/>
  F : PMIOPort  Side=Left
  connections:
  Solid/RConn1 -- ReferenceFrame/RConn1 -- F/RConn1

== system FBR25_model_4_rotating_tyres_with_ground_no_contact/FBR25_VD_1_RIGID/FBR25_VD_0300_STEERING_Computurtle_3_1_RIGID/FBR25_VD_33_00_1_RIGID/FBR25_VD_33_01_1_RIGID/PART_STEERING_RACK_MOUNT_with_added_points_2_RIGID ==
  ReferenceFrame : sm_lib/Frames and Transforms/Reference Frame
  Solid : sm_lib/Body Elements/File Solid  ExtGeomFileName=PART - STEERING RACK MOUNT with added points_Default_sldprt.STEP  UnitType=FromFile  ExtGeomFileUnits=m  StepReaderType=HEX  ExportConvexHullGeometry=off  InertiaType=Custom  BasedOnType=DensityFromFile  Density=1000  DensityUnits=kg/m^3  Mass=smiData.Solid(92).mass  MassUnits=kg  CenterOfMass=smiData.Solid(92).CoM  CenterOfMassUnits=mm  MomentsOfInertia=smiData.Solid(92).MoI  MomentsOfInertiaUnits=kg*mm^2  ProductsOfInertia=smiData.Solid(92).PoI  ProductsOfInertiaUnits=kg*mm^2  GraphicType=FromGeometry  MarkerShape=Sphere  MarkerSize=10  GraphicVisPropType=SimpleVisualProperties  GraphicDiffuseColor=smiData.Solid(92).color  GraphicOpacity=smiData.Solid(92).opacity  GraphicSpecularColor=[0.5 0.5 0.5 1.0]  GraphicAmbientColor=[0.15 0.15 0.15 1.0]  GraphicEmissiveColor=[0.0 0.0 0.0 1.0]  GraphicShininess=75  DoExposeReferenceFrame=on  SerializedFrames=<Frames/>
  F : PMIOPort  Side=Left
  connections:
  Solid/RConn1 -- ReferenceFrame/RConn1 -- F/RConn1

== system FBR25_model_4_rotating_tyres_with_ground_no_contact/FBR25_VD_1_RIGID/FBR25_VD_0300_STEERING_Computurtle_3_1_RIGID/FBR25_VD_33_00_1_RIGID/FBR25_VD_33_01_1_RIGID/PART_STEERING_RACK_MOUNT_with_added_points_3_RIGID ==
  ReferenceFrame : sm_lib/Frames and Transforms/Reference Frame
  Solid : sm_lib/Body Elements/File Solid  ExtGeomFileName=PART - STEERING RACK MOUNT with added points_Default_sldprt.STEP  UnitType=FromFile  ExtGeomFileUnits=m  StepReaderType=HEX  ExportConvexHullGeometry=off  InertiaType=Custom  BasedOnType=DensityFromFile  Density=1000  DensityUnits=kg/m^3  Mass=smiData.Solid(92).mass  MassUnits=kg  CenterOfMass=smiData.Solid(92).CoM  CenterOfMassUnits=mm  MomentsOfInertia=smiData.Solid(92).MoI  MomentsOfInertiaUnits=kg*mm^2  ProductsOfInertia=smiData.Solid(92).PoI  ProductsOfInertiaUnits=kg*mm^2  GraphicType=FromGeometry  MarkerShape=Sphere  MarkerSize=10  GraphicVisPropType=SimpleVisualProperties  GraphicDiffuseColor=smiData.Solid(92).color  GraphicOpacity=smiData.Solid(92).opacity  GraphicSpecularColor=[0.5 0.5 0.5 1.0]  GraphicAmbientColor=[0.15 0.15 0.15 1.0]  GraphicEmissiveColor=[0.0 0.0 0.0 1.0]  GraphicShininess=75  DoExposeReferenceFrame=on  SerializedFrames=<Frames/>
  F : PMIOPort  Side=Left
  connections:
  Solid/RConn1 -- ReferenceFrame/RConn1 -- F/RConn1

== system FBR25_model_4_rotating_tyres_with_ground_no_contact/FBR25_VD_1_RIGID/FBR25_VD_0300_STEERING_Computurtle_3_1_RIGID/FBR25_VD_33_00_1_RIGID/FBR25_VD_33_01_1_RIGID/PART_STEERING_RACK_MOUNT_with_added_points_4_RIGID ==
  ReferenceFrame : sm_lib/Frames and Transforms/Reference Frame
  Solid : sm_lib/Body Elements/File Solid  ExtGeomFileName=PART - STEERING RACK MOUNT with added points_Default_sldprt.STEP  UnitType=FromFile  ExtGeomFileUnits=m  StepReaderType=HEX  ExportConvexHullGeometry=off  InertiaType=Custom  BasedOnType=DensityFromFile  Density=1000  DensityUnits=kg/m^3  Mass=smiData.Solid(92).mass  MassUnits=kg  CenterOfMass=smiData.Solid(92).CoM  CenterOfMassUnits=mm  MomentsOfInertia=smiData.Solid(92).MoI  MomentsOfInertiaUnits=kg*mm^2  ProductsOfInertia=smiData.Solid(92).PoI  ProductsOfInertiaUnits=kg*mm^2  GraphicType=FromGeometry  MarkerShape=Sphere  MarkerSize=10  GraphicVisPropType=SimpleVisualProperties  GraphicDiffuseColor=smiData.Solid(92).color  GraphicOpacity=smiData.Solid(92).opacity  GraphicSpecularColor=[0.5 0.5 0.5 1.0]  GraphicAmbientColor=[0.15 0.15 0.15 1.0]  GraphicEmissiveColor=[0.0 0.0 0.0 1.0]  GraphicShininess=75  DoExposeReferenceFrame=on  SerializedFrames=<Frames/>
  F : PMIOPort  Side=Left
  connections:
  Solid/RConn1 -- ReferenceFrame/RConn1 -- F/RConn1

== system FBR25_model_4_rotating_tyres_with_ground_no_contact/FBR25_VD_1_RIGID/FBR25_VD_0300_STEERING_Computurtle_3_1_RIGID/FBR25_VD_33_00_1_RIGID/FBR25_VD_33_01_1_RIGID/PART_STEERING_RACK_SHAFT_with_added_points_1_RIGID ==
  ReferenceFrame : sm_lib/Frames and Transforms/Reference Frame
  Solid : sm_lib/Body Elements/File Solid  ExtGeomFileName=PART - STEERING RACK SHAFT with added points_Default_sldprt.STEP  UnitType=FromFile  ExtGeomFileUnits=m  StepReaderType=HEX  ExportConvexHullGeometry=off  InertiaType=Custom  BasedOnType=DensityFromFile  Density=1000  DensityUnits=kg/m^3  Mass=smiData.Solid(93).mass  MassUnits=kg  CenterOfMass=smiData.Solid(93).CoM  CenterOfMassUnits=mm  MomentsOfInertia=smiData.Solid(93).MoI  MomentsOfInertiaUnits=kg*mm^2  ProductsOfInertia=smiData.Solid(93).PoI  ProductsOfInertiaUnits=kg*mm^2  GraphicType=FromGeometry  MarkerShape=Sphere  MarkerSize=10  GraphicVisPropType=SimpleVisualProperties  GraphicDiffuseColor=smiData.Solid(93).color  GraphicOpacity=smiData.Solid(93).opacity  GraphicSpecularColor=[0.5 0.5 0.5 1.0]  GraphicAmbientColor=[0.15 0.15 0.15 1.0]  GraphicEmissiveColor=[0.0 0.0 0.0 1.0]  GraphicShininess=75  DoExposeReferenceFrame=on  SerializedFrames=<Frames/>
  F : PMIOPort  Side=Left
  connections:
  Solid/RConn1 -- ReferenceFrame/RConn1 -- F/RConn1
